simulink model "LuGre_micro_sinewave"  (R2026a)
settings: Solver=ode23tb  MaxStep=1e-4  RelTol=1e-7  AbsTol=1e-10
model workspace (MAT data in the model file):
  omega = Simulink.Parameter
  omega.Value = 25
  omega.Complexity = 'real'
  omega.Dimensions = [1 1]
  omega.DataType = 'auto'
undefined symbols (not defined in the file): amp, w
settings Model: Creator=shuki  LastModifiedBy=shuki

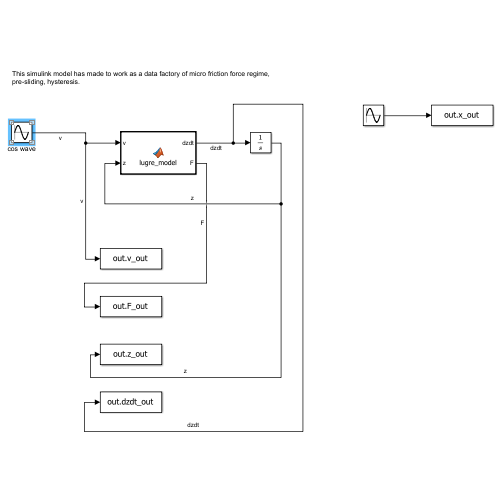
[thumbnail: Simulink's stored preview of the top-level diagram]
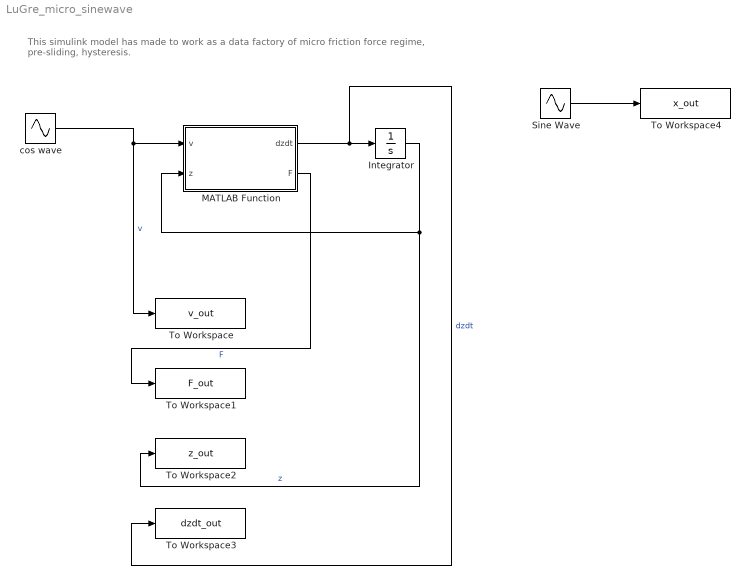
== system LuGre_micro_sinewave ==
  note: This simulink model has made to work as a data factory of micro friction force regime, pre-sliding, hysteresis.
  Integrator : Integrator
  MATLAB Function : MATLAB Function  TreatAsAtomicUnit=on
  Sine Wave : Sin  Amplitude=amp  Frequency=w  SampleTime=0
  To Workspace : ToWorkspace  VariableName=v_out  SaveFormat=Timeseries  SampleTime=-1
  To Workspace1 : ToWorkspace  VariableName=F_out  SaveFormat=Timeseries  SampleTime=-1
  To Workspace2 : ToWorkspace  VariableName=z_out  SaveFormat=Timeseries  SampleTime=-1
  To Workspace3 : ToWorkspace  VariableName=dzdt_out  SaveFormat=Timeseries  SampleTime=-1
  To Workspace4 : ToWorkspace  VariableName=x_out  SaveFormat=Timeseries  SampleTime=-1
  cos wave : Sin  Amplitude=amp * w  Frequency=w  Phase=pi/2  SampleTime=0
  wires:
  Integrator/1 -> To Workspace2/1, MATLAB Function/2(z)  "z"
  MATLAB Function/1(dzdt) -> To Workspace3/1, Integrator/1  "dzdt"
  cos wave/1 -> To Workspace/1, MATLAB Function/1(v)  "v"
  MATLAB Function/2(F) -> To Workspace1/1  "F"
  Sine Wave/1 -> To Workspace4/1

== matlab function LuGre_micro_sinewave/MATLAB Function ==
  data: v input; dzdt output; z input; F output
%function [dzdt, F] = lugre_model(v, z, sigma0, sigma1, sigma2, Fc, Fs, vs)
function [dzdt, F] = lugre_model(v, z)
    % parameters (from the table I in the paper of LuGre) 
    sigma0 = 1e5; % stiffness, refined
    sigma1 = sqrt(sigma0); % damping(減衰)
    sigma2 = 0.4; % viscosity coefficient(粘性係数)
    Fc = 1.0; % dynamic friction force(動摩擦力)
    Fs = 1.5; % static friction force(静止摩擦力)
    vs = 0.001; % stribeck speed(ストライベック速度)
    
    % g(v)
    gv = Fc + (Fs - Fc) * exp(-(v/vs)^2);
    
    % dz/dt
    dzdt = v - (sigma0 * abs(v) / gv) * z;
    
    % F
    F = sigma0 * z + sigma1 * dzdt + sigma2 * v;
end
